simulink model "Wind_PMSG_Transient_R3"  (R2026a)
settings: Solver=ode15s  StopTime=Base.Simulation.StopTime  MaxStep=Base.Simulation.MaxStep
InitFcn:
  | root=fileparts(fileparts(get_param(bdroot,'FileName'))); run(fullfile(root,'parameters','init_wind_pmsg_transient_r3.m'));
undefined symbols (not defined in the file): Base, Control, Converter, Drive, Filter, Grid, PMSG, Wind
libraries: nesl_utility x14, ee_lib x12, fl_lib x4, simulink x2
(part 2 of 2)

== system Wind_PMSG_Transient_R3/04 GFL Control and SPWM/02 Synchronization SRF-PLL/Park Voltage ==
  alpha beta : Inport
  theta : Inport  Port=2
  Separate alpha beta : Demux  Outputs=2
  alpha cos : Product
  alpha sin : Product
  beta cos : Product
  beta sin : Product
  cos theta : Trigonometry  Operator=cos
  d = alpha cos + beta sin : Sum
  dq vector : Mux  Inputs=2
  q = -alpha sin + beta cos : Sum  Inputs=-+
  sin theta : Trigonometry
  dq : Outport
  wires:
  alpha beta/1 -> Separate alpha beta/1
  theta/1 -> cos theta/1, sin theta/1
  Separate alpha beta/1 -> alpha cos/1, alpha sin/1
  cos theta/1 -> alpha cos/2, beta cos/2
  Separate alpha beta/2 -> beta sin/1, beta cos/1
  sin theta/1 -> beta sin/2, alpha sin/2
  alpha cos/1 -> d = alpha cos + beta sin/1
  beta sin/1 -> d = alpha cos + beta sin/2
  alpha sin/1 -> q = -alpha sin + beta cos/1
  beta cos/1 -> q = -alpha sin + beta cos/2
  d = alpha cos + beta sin/1 -> dq vector/1
  q = -alpha sin + beta cos/1 -> dq vector/2
  dq vector/1 -> dq/1

== system Wind_PMSG_Transient_R3/04 GFL Control and SPWM/03 DC Voltage and Current Reference/Park Voltage ==
  alpha beta : Inport
  theta : Inport  Port=2
  Separate alpha beta : Demux  Outputs=2
  alpha cos : Product
  alpha sin : Product
  beta cos : Product
  beta sin : Product
  cos theta : Trigonometry  Operator=cos
  d : Sum
  dq vector : Mux  Inputs=2
  q : Sum  Inputs=-+
  sin theta : Trigonometry
  dq : Outport
  wires:
  alpha beta/1 -> Separate alpha beta/1
  theta/1 -> cos theta/1, sin theta/1
  Separate alpha beta/1 -> alpha cos/1, alpha sin/1
  cos theta/1 -> alpha cos/2, beta cos/2
  Separate alpha beta/2 -> beta sin/1, beta cos/1
  sin theta/1 -> beta sin/2, alpha sin/2
  alpha cos/1 -> d/1
  beta sin/1 -> d/2
  alpha sin/1 -> q/1
  beta cos/1 -> q/2
  d/1 -> dq vector/1
  q/1 -> dq vector/2
  dq vector/1 -> dq/1

== system Wind_PMSG_Transient_R3/04 GFL Control and SPWM/05 dq Current Controller/Inverse Park and Clarke ==
  dq : Inport
  theta : Inport  Port=2
  Inverse Clarke : Gain  Gain=sqrt(2/3)*[1 -0.5 -0.5;0 sqrt(3)/2 -sqrt(3)/2]  Multiplication=Matrix(u*K)
  Separate dq : Demux  Outputs=2
  alpha : Sum  Inputs=+-
  alpha beta : Mux  Inputs=2
  beta : Sum
  cos theta : Trigonometry  Operator=cos
  d cos : Product
  d sin : Product
  q cos : Product
  q sin : Product
  sin theta : Trigonometry
  abc : Outport
  wires:
  dq/1 -> Separate dq/1
  theta/1 -> cos theta/1, sin theta/1
  Separate dq/1 -> d cos/1, d sin/1
  cos theta/1 -> d cos/2, q cos/2
  Separate dq/2 -> q sin/1, q cos/1
  sin theta/1 -> q sin/2, d sin/2
  d cos/1 -> alpha/1
  q sin/1 -> alpha/2
  d sin/1 -> beta/1
  q cos/1 -> beta/2
  alpha/1 -> alpha beta/1
  beta/1 -> alpha beta/2
  alpha beta/1 -> Inverse Clarke/1
  Inverse Clarke/1 -> abc/1

== system Wind_PMSG_Transient_R3/04 GFL Control and SPWM/05 dq Current Controller/Park Current ==
  alpha beta : Inport
  theta : Inport  Port=2
  Separate alpha beta : Demux  Outputs=2
  alpha cos : Product
  alpha sin : Product
  beta cos : Product
  beta sin : Product
  cos theta : Trigonometry  Operator=cos
  d : Sum
  dq vector : Mux  Inputs=2
  q : Sum  Inputs=-+
  sin theta : Trigonometry
  dq : Outport
  wires:
  alpha beta/1 -> Separate alpha beta/1
  theta/1 -> cos theta/1, sin theta/1
  Separate alpha beta/1 -> alpha cos/1, alpha sin/1
  cos theta/1 -> alpha cos/2, beta cos/2
  Separate alpha beta/2 -> beta sin/1, beta cos/1
  sin theta/1 -> beta sin/2, alpha sin/2
  alpha cos/1 -> d/1
  beta sin/1 -> d/2
  alpha sin/1 -> q/1
  beta cos/1 -> q/2
  d/1 -> dq vector/1
  q/1 -> dq vector/2
  dq vector/1 -> dq/1

== system Wind_PMSG_Transient_R3/04 GFL Control and SPWM/05 dq Current Controller/Park Voltage ==
  alpha beta : Inport
  theta : Inport  Port=2
  Separate alpha beta : Demux  Outputs=2
  alpha cos : Product
  alpha sin : Product
  beta cos : Product
  beta sin : Product
  cos theta : Trigonometry  Operator=cos
  d : Sum
  dq vector : Mux  Inputs=2
  q : Sum  Inputs=-+
  sin theta : Trigonometry
  dq : Outport
  wires:
  alpha beta/1 -> Separate alpha beta/1
  theta/1 -> cos theta/1, sin theta/1
  Separate alpha beta/1 -> alpha cos/1, alpha sin/1
  cos theta/1 -> alpha cos/2, beta cos/2
  Separate alpha beta/2 -> beta sin/1, beta cos/1
  sin theta/1 -> beta sin/2, alpha sin/2
  alpha cos/1 -> d/1
  beta sin/1 -> d/2
  alpha sin/1 -> q/1
  beta cos/1 -> q/2
  d/1 -> dq vector/1
  q/1 -> dq vector/2
  dq vector/1 -> dq/1
